simulink model "lab2_model"  (R2026b)
settings: Solver=VariableStepAuto
settings Model: Creator=Anna  LastModifiedBy=Anna

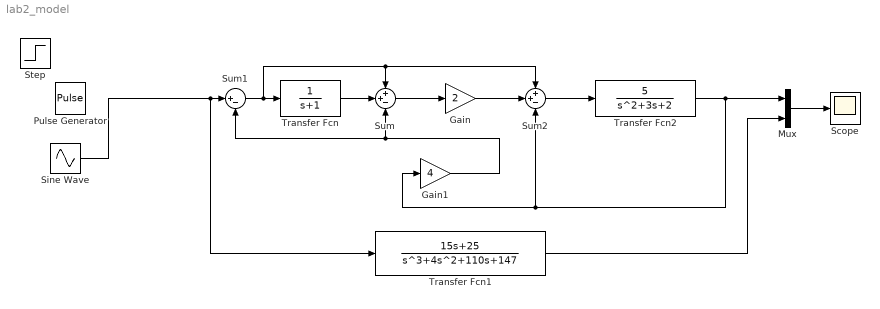
== system lab2_model ==
  Gain : Gain  Gain=2
  Gain1 : Gain  Gain=4
  Mux : Mux  Inputs=2
  Pulse Generator : DiscretePulseGenerator  PulseType=Time based  Period=10  PulseWidth=5
  Scope : Scope
      settings: ActiveDisplayYMinimum=-0.43289554872470504  ActiveDisplayYMaximum=0.3304034293304407
  Sine Wave : Sin  SampleTime=0
  Step : Step  SampleTime=0
  Sum : Sum  Inputs=++-
  Sum1 : Sum  Inputs=|+-
  Sum2 : Sum  Inputs=++-
  Transfer Fcn : TransferFcn  Denominator=[1 1]
  Transfer Fcn1 : TransferFcn  Numerator=[15 25]  Denominator=[1 4 110 147]
  Transfer Fcn2 : TransferFcn  Numerator=[5]  Denominator=[1 3 2]
  wires:
  Mux/1 -> Scope/1
  Gain1/1 -> Sum/3, Sum1/2
  Sum1/1 -> Transfer Fcn/1, Sum2/1, Sum/1
  Transfer Fcn/1 -> Sum/2
  Sum/1 -> Gain/1
  Gain/1 -> Sum2/2
  Sum2/1 -> Transfer Fcn2/1
  Transfer Fcn2/1 -> Sum2/3, Gain1/1, Mux/1
  Sine Wave/1 -> Transfer Fcn1/1, Sum1/1
  Transfer Fcn1/1 -> Mux/2
